simulink model "controller_V1"  (R2025b)
settings: Solver=VariableStepAuto  StartTime=0.0  StopTime=10.0  RelTol=1e-3
undefined symbols (not defined in the file): k_drag, rr_stop_dest
libraries: simulink x3
settings Model: Creator=AORUS  LastModifiedBy=AORUS

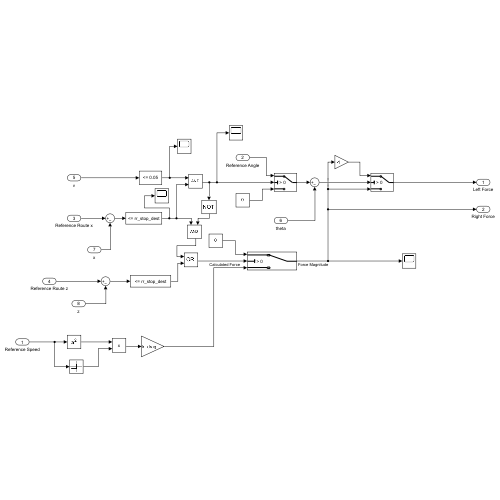
[thumbnail: Simulink's stored preview of the top-level diagram]
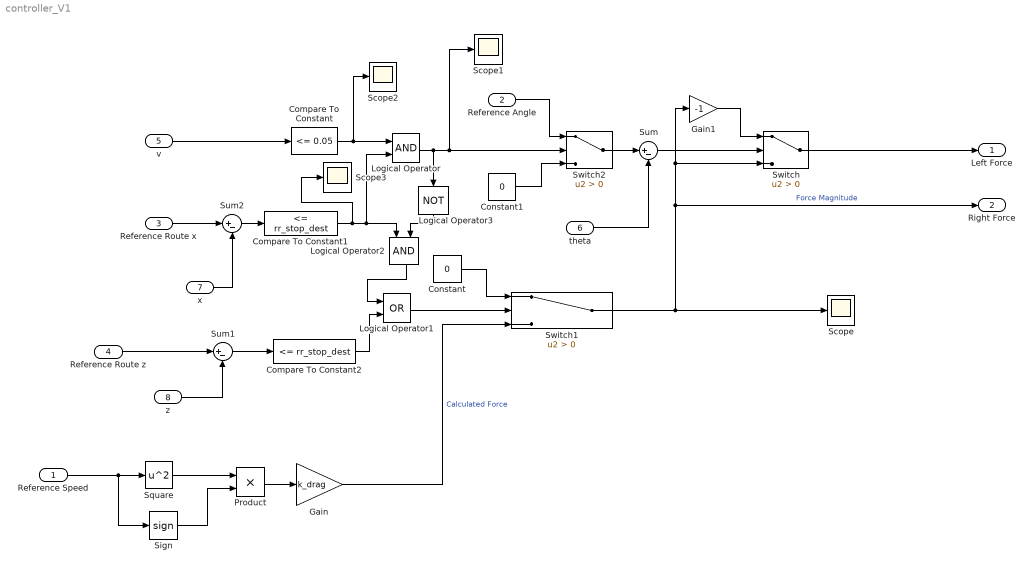
== system controller_V1 ==
  Reference Speed : Inport
  Reference Angle : Inport  Port=2
  Reference Route x : Inport  Port=3
  Reference Route z : Inport  Port=4
  v : Inport  Port=5
  theta : Inport  Port=6
  x : Inport  Port=7
  z : Inport  Port=8
  Compare To Constant : simulink/Logic and Bit Operations/Compare To Constant  relop=<=  const=0.05  OutDataTypeStr=boolean
  Compare To Constant1 : simulink/Logic and Bit Operations/Compare To Constant  relop=<=  const=rr_stop_dest  OutDataTypeStr=boolean
  Compare To Constant2 : simulink/Logic and Bit Operations/Compare To Constant  relop=<=  const=rr_stop_dest  OutDataTypeStr=boolean
  Constant : Constant  Value=0
  Constant1 : Constant  Value=0
  Gain : Gain  Gain=k_drag
  Gain1 : Gain  Gain=-1
  Logical Operator : Logic  AllPortsSameDT=off  OutDataTypeStr=boolean
  Logical Operator1 : Logic  Operator=OR  AllPortsSameDT=off  OutDataTypeStr=boolean
  Logical Operator2 : Logic  AllPortsSameDT=off  OutDataTypeStr=boolean
  Logical Operator3 : Logic  Operator=NOT  AllPortsSameDT=off  OutDataTypeStr=boolean
  Product : Product
  Scope{,1..3} (4 alike) : Scope
      Scope settings: ActiveDisplayYMinimum=0.872  ActiveDisplayYMaximum=1.072
      Scope1 settings: ActiveDisplayYMinimum=-0.125  ActiveDisplayYMaximum=1.125
      Scope2 settings: ActiveDisplayYMinimum=-0.125  ActiveDisplayYMaximum=1.125  DataLoggingVariableName=ScopeData2
      Scope3 settings: ActiveDisplayYMinimum=-0.125  ActiveDisplayYMaximum=1.125  DataLoggingVariableName=ScopeData3
  Sign : Signum
  Square : Math  Operator=square
  Sum : Sum  Inputs=|+-
  Sum1 : Sum  Inputs=|+-
  Sum2 : Sum  Inputs=|+-
  Switch : Switch  Criteria=u2 > Threshold  SaturateOnIntegerOverflow=off  InputSameDT=off
  Switch1 : Switch  Criteria=u2 > Threshold  SaturateOnIntegerOverflow=off  InputSameDT=off
  Switch2 : Switch  Criteria=u2 > Threshold  SaturateOnIntegerOverflow=off  InputSameDT=off
  Left Force : Outport
  Right Force : Outport  Port=2
  wires:
  Constant1/1 -> Switch2/3
  Compare To Constant2/1 -> Logical Operator1/2
  theta/1 -> Sum/2
  Reference Route z/1 -> Sum1/1
  Reference Route x/1 -> Sum2/1
  Compare To Constant/1 -> Scope2/1, Logical Operator/1
  Gain1/1 -> Switch/1
  x/1 -> Sum2/2
  Switch/1 -> Left Force/1
  Logical Operator/1 -> Logical Operator3/1, Scope1/1, Switch2/2
  Reference Angle/1 -> Switch2/1
  Switch1/1 -> Scope/1, Right Force/1, Switch/3, Gain1/1  "Force Magnitude"
  Logical Operator1/1 -> Switch1/2
  Sum/1 -> Switch/2
  Logical Operator2/1 -> Logical Operator1/1
  Sign/1 -> Product/2
  Gain/1 -> Switch1/3  "Calculated Force"
  Product/1 -> Gain/1
  z/1 -> Sum1/2
  Compare To Constant1/1 -> Scope3/1, Logical Operator/2, Logical Operator2/1
  Square/1 -> Product/1
  Switch2/1 -> Sum/1
  Sum2/1 -> Compare To Constant1/1
  Constant/1 -> Switch1/1
  Logical Operator3/1 -> Logical Operator2/2
  v/1 -> Compare To Constant/1
  Sum1/1 -> Compare To Constant2/1
  Reference Speed/1 -> Sign/1, Square/1
